simulink library "ASEToolBox2023a"  (R2023a)
settings: Solver=ode45  StartTime=0.0  StopTime=10.0  RelTol=1e-3  EnableMultiTasking=on
values from neighbouring files (symbols this model uses):
  dt = get_param(gcbh, 'g_output_datatype')    [maskSysComCallbacks_Receive.m]    (also in maskSysComCallbacks_Send.m = get_param(gcbh, 'g_input_datatype'))
undefined symbols (not defined in the file or in its folder): dCx, dCy, dCz, DiscIntNeverNeededParam, Discrete, dmassX, dmassY, dmassZ, dMx, dMy, dMz, dp, dp0, dp1, dp2, dp3, lmd_high, lmd_low, magnitude, Newton, p0, p1, p2, p3, p4, phi0, phi000, phi1, phi2, phi3, phi4, r1, r2, r3, r4, Raphson, theta0, theta1, theta2, theta3, theta4, Time, u0, u1, u2, u3, v0, v0_max, v0_min, v1, v111, v2, v222, v3, v333, v4, W1, w1, w2, W2 ... (+2)
libraries: simulink x38, etargetslib x28, simulink_extras x5, slpidlib x2, ctrlSharedLib x2, aerolibatmos2 x1, aerolibconvert2 x1, aerolibtransform2 x1, sharedtransform x1, dspstat3 x1, dspsolvers x1
(part 1 of 6)
settings Model: Creator=sunzx.fnst  LastModifiedBy=zqhkd
settings SolverCC: AlgebraicLoopSolver=TrustRegion
settings DataIOCC: LimitDataPoints=on  SaveFormat=Array  ReturnWorkspaceOutputs=off
settings OptimizationCC: LifeSpan=inf
settings DebuggingCC: UnderspecifiedInitializationDetection=Classic  MergeDetectMultiDrivingBlocksExec=none  SolverPrmCheckMsg=warning  UnconnectedInputMsg=warning  UnconnectedOutputMsg=warning  UnconnectedLineMsg=warning  SFUnexpectedBacktrackingDiag=warning  SFNoUnconditionalDefaultTransitionDiag=warning  SFExecutionAtInitializationDiag=none  ArithmeticOperatorsInVariantConditions=warning
settings HardwareCC: ProdBitPerPointer=32  ProdBitPerSizeT=32  ProdBitPerPtrDiffT=32  ProdLargestAtomicFloat=None  ProdIntDivRoundTo=Undefined  ProdEndianess=Unspecified  ProdWordSize=32  ProdHWDeviceType=32-bit Generic
settings ModelReferenceCC: PropagateSignalLabelsOutOfModel=off
settings SFSimCC: SimUseLocalCustomCode=off  CustomCodeUndefinedFunction=UseInterfaceOnly
settings RTWCC: RTWUseLocalCustomCode=off
settings CodeAppCC: StateflowObjectComments=on
settings GRTTargetCC: TargetLangStandard=C89/C90 (ANSI)
settings ConfigComp: CovMetricSettings=dw  CovSaveCumulativeToWorkspaceVar=on  CovSaveSingleToWorkspaceVar=on  CovExternalEMLEnable=off  CovSFcnEnable=off  CovBoundaryAbsTol=1.0e-5

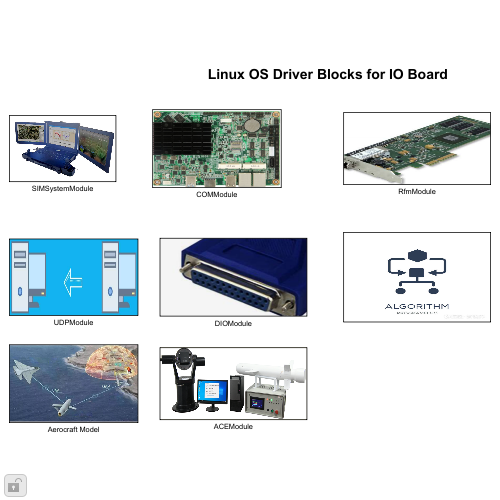
[thumbnail: Simulink's stored preview of the top-level diagram]
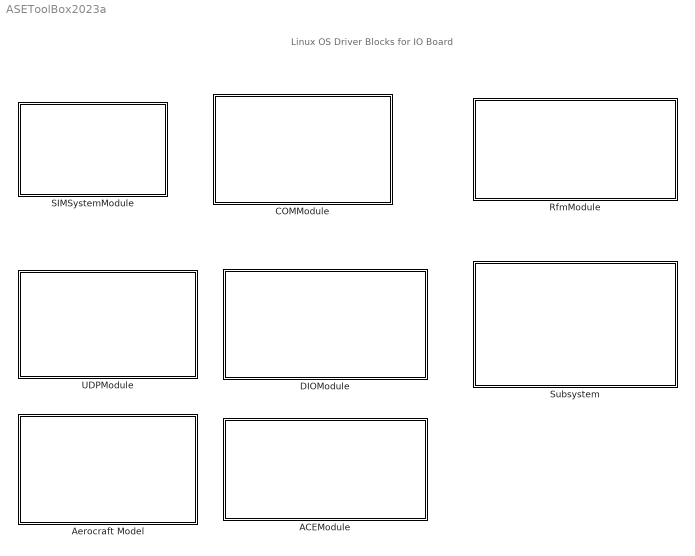
== system ASEToolBox2023a ==
  note: Linux OS Driver Blocks for IO Board
  ACEModule : Subsystem
      mask Display: image('ACEModule.png');
  Aerocraft Model : Subsystem
      mask Display: image('ASEApp.png');
  COMModule : Subsystem
      mask Display: image('MainBoardCom.png'); % 使用工具条上的 "编辑图像" 进行更改。
  DIOModule : Subsystem
      mask Display: image('parport.png'); % 使用工具条上的 "编辑图像" 进行更改。
  RfmModule : Subsystem
      mask Display: image('GE5565.png'); % 使用工具条上的 "编辑图像" 进行更改。
  SIMSystemModule : Subsystem
      mask Display: image('ASESystem.jpg'); % 使用工具条上的 "编辑图像" 进行更改。
  Subsystem : Subsystem
      mask Display: image('Algorithm.jpg'); % 使用工具条上的 "编辑图像" 进行更改。
  UDPModule : Subsystem
      mask Display: image('UDP.png'); % 使用工具条上的 "编辑图像" 进行更改。

== system ASEToolBox2023a/ACEModule ==
  IMU : Subsystem
  ServoCardPack : Subsystem  mask{g_FrameType=80, g_SendId=0}
      mask prompts: g_FrameType "请输入帧类型码："; g_SendId "发送方ID:"
      mask DialogControl ParameterGroupVar Prompt: 参数
  ServoCardUnpack : Subsystem
  TurnTable : Subsystem

== system ASEToolBox2023a/Aerocraft Model ==
  ACE Aerodynamic for 3DOF : Subsystem  mask(ACE Aerodynamic for 3DOF){}
      mask help: There is ACE Aerodynamic for 3DOF Model, including the ACE aircraft's aerodynamic force efficient models, and it is employed to simulate the 3DOF motion.
      mask Display:
      | %image(imread('aeroaerodynamics.bmp','bmp'),'center')
      | port_label('input',1,'Mach(M)','texmode','on');
      | port_label('input',2,'abv(deg)','texmode','on');
      | port_label('output',1,'Cxyz','texmode','on');
  ACE Aerodynamic for 6DOF : Subsystem  mask(ACE Aerodynamic for 6DOF){}
      mask help: There is ACE Aerodynamic for 6DOF Model, including the ACE aircraft's aerodynamic force efficient models and aerodynamic moment efficient models, and it is employed to simulate the 6DOF motion.
      mask Display:
      | %image(imread('aeroaerodynamics.bmp','bmp'),'center')
      | port_label('input',1,'Mach(M)','texmode','on');
      | port_label('input',2,'abv(deg)','texmode','on');
      | port_label('input',3,'WXYZ','texmode','on');
      | port_label('input',4,'Deltaxyz(deg)','texmode','on');
      | port_label('output',1,'Cxyz','texmode','on');
      | port_label('output',2,'mxyz','texmode','on');
  ACE Equation of 6DOF's Motion : Subsystem  mask(Equation of 6DOF's  Motion){}
      mask help: There is Equation of 6DOF Motion Model.
  ACE Guidance and Control Algorithm : Subsystem
  ACE Mass : Subsystem  mask(ACE Mass Properties){}
      mask help: There is ACE Mass Properties Model.
      mask Display:
      | %image(imread('aeromassprop.bmp','bmp'),'center');
      | port_label('input',1,'Time(s)','texmode','on');
      | port_label('output',1,'Mass(kg)','texmode','on');
  ACE Propulsion : Subsystem  mask(ACE Propulsion){}
      mask help: There is ACE Propulsion Model.
      mask Display:
      | %image(imread('aeropropulsion.bmp','bmp'),'center')
      | port_label('input',1,'Time(s)','texmode','on');
      | port_label('output',1,'P(N)','texmode','on');

== system ASEToolBox2023a/COMModule ==
  XComIn : S-Function  FunctionName=readXComAPI  Parameters=g_serial_select,g_baudrate, g_parity, g_databit, g_stopbit, g_data_size, g_sample_time  SFunctionDeploymentMode=off  EnableBusSupport=off  mask(CP-116E-A接收模块){g_serial_select=ttyMUE0, g_baudrate=460800, g_parity=None, g_databit=8, g_stopbit=1, g_data_size=1, g_sample_time=-1}
      mask prompts: g_serial_select "串口号："; g_baudrate "波特率："; g_parity "校验位："; g_databit "数据位："; g_stopbit "停止位："; g_data_size "帧长度："; g_sample_time "采样时间："
      mask help:
      | 多串口中选择串口号的数据接收模块。
      | 用户需要指定串口设备号、接收数据的数据类型和长度。
      | 串口接收模块有两个输出端口，第一个端口输出串口上发来被接收到的数据，并转换为用户设定的数据类型发出；
      | 第二个端口Len表示每个步长下所接收到的数据长度，用于帮助用户分析和对数据进行后处理。
      mask Help: https://moxa.com.cn/products/industrial-edge-connectivity/multiport-serial-boards/pcie-upci-pci-serial-cards/cp-116e-a
      mask TypeOptions g_serial_select: ttyS0 | ttyS1 | ttyS2 | ttyS3 | ttyS4 | ttyS5 | ttyS6 | ttyMUE0 | ttyMUE1 | ttyMUE2 | ttyMUE3 | ttyMUE4 | ttyMUE5 | ttyMUE6 | ttyMUE7 | ttyMUE8 | ttyMUE9 | ttyMUE10 | ttyMUE11 | ttyMUE12 | ttyMUE13 | ttyMUE14 | ttyMUE15 | ttyUSB0 | ttyUSB1 | ttyUSB2 | ttyUSB3 | Custom
      mask TypeOptions g_baudrate: 921600 | 576000 | 500000 | 460800 | 230400 | 115200 | 57600 | 38400 | 19200 | 9600 | Custom
      mask TypeOptions g_parity: None | Odd | Even | Mark | Space
      mask DialogControl ParameterGroupVar Prompt: ASE仿真系统串口接收模块
      mask Display:
      | color('blue');
      | serialDevice = get_param(gcbh, 'g_serial_select');
      | port_label('output', 1, serialDevice);
      | image('MainBoardCom.png', [0 0 0.33 0.48]);
  XComOut : S-Function  FunctionName=writeXComAPI  Parameters=g_serial_select,g_baudrate, g_parity, g_databit, g_stopbit,g_sample_time  SFunctionDeploymentMode=off  EnableBusSupport=off  mask(CP-116E-A发送模块){g_serial_select=ttyMUE0, g_baudrate=460800, g_parity=None, g_databit=8, g_stopbit=1, g_sample_time=-1}
      mask prompts: g_serial_select "串口号："; g_baudrate "波特率："; g_parity "校验位："; g_databit "数据位："; g_stopbit "停止位："; g_sample_time "采样时间："
      mask help: 根据用户设置的串口号，指定的数据类型，将数据对外部进行发送的模块。
      mask Help: https://moxa.com.cn/products/industrial-edge-connectivity/multiport-serial-boards/pcie-upci-pci-serial-cards/cp-116e-a
      mask TypeOptions g_serial_select: ttyS0 | ttyS1 | ttyS2 | ttyS3 | ttyS4 | ttyS5 | ttyS6 | ttyMUE0 | ttyMUE1 | ttyMUE2 | ttyMUE3 | ttyMUE4 | ttyMUE5 | ttyMUE6 | ttyMUE7 | ttyMUE8 | ttyMUE9 | ttyMUE10 | ttyMUE11 | ttyMUE12 | ttyMUE13 | ttyMUE14 | ttyMUE15 | ttyUSB0 | ttyUSB1 | ttyUSB2 | ttyUSB3 | Custom
      mask TypeOptions g_baudrate: 921600 | 576000 | 500000 | 460800 | 230400 | 115200 | 57600 | 38400 | 19200 | 9600 bps
      mask TypeOptions g_parity: None | Odd | Even | Mark | Space
      mask DialogControl ParameterGroupVar Prompt: ASE仿真串口发送模块
      mask Display:
      | color('blue');
      | serialDevice = get_param(gcbh, 'g_serial_select');
      | port_label('input', 1, serialDevice);
      | image('MainBoardCom.png', [0.67 0 1.0 0.48]);

== system ASEToolBox2023a/DIOModule ==
  ParPortRead : S-Function  FunctionName=ParPortDataRead  Parameters=g_par_select, g_ext_trigger, g_pin  SFunctionDeploymentMode=off  EnableBusSupport=off  mask(Linux工控机主板并口设备){g_par_select=/dev/parport0, g_ext_trigger=on, g_pin=PIN15 (S3)}
      mask prompts: g_par_select "并口设备号:"; g_ext_trigger "外部时钟源触发:"; g_pin "时钟源PIN:"
      mask help: 此模块将输出Linux IPC并口设备的数据寄存器的值。数据寄存器包括D7|D6|D5|D4|D3|D2|D1|D0总共8个数据位，合并位uint8类型输出。
      mask TypeOptions g_par_select: /dev/parport0
      mask TypeOptions g_pin: PIN15 (S3) | PIN13 (S4) | PIN12 (S5) | PIN10 (S6) | PIN11 (S7)
      mask DialogControl ParameterGroupVar Prompt: 工控机主板板载并口管理
      mask DialogControl Control1 Prompt: 此模块将输出工控机主板并口设备DB25输入引脚高低电平状态。各引脚和输入寄存器位之间关系如下：
      mask DialogControl Control3 Prompt: P15--Di3, P13--Di4, P12--Di5, P10--Di6, P11--Di7
      mask DialogControl g_pin Tooltip: 并口DB25引脚定义
      mask Display:
      | warning off;
      | image('parport.png');
      | ext_trigger = get_param(gcbh, 'g_ext_trigger');
      | pin = get_param(gcbh, 'g_pin');
      | if strcmp(ext_trigger, 'off')
      |     color('cyan');
      |     port_label('output', 1, 'data');
      | else
      |     color('cyan');
      |     disp(['外部时钟源:' pin]);
      | end
  ParPortWrite : S-Function  FunctionName=ParPortDataWrite  Parameters=g_par_select  SFunctionDeploymentMode=off  EnableBusSupport=off  mask(Linux工控机主板并口设备){g_par_select=/dev/parport0}
      mask prompts: g_par_select "并口号:"
      mask help: 此模块将模型输入值写入到Linux IPC并口设备的数据寄存器。数据寄存器包括D7|D6|D5|D4|D3|D2|D1|D0总共8个数据位，模型中将8个bit合并为uint8类型输入。
      mask TypeOptions g_par_select: /dev/parport0
      mask DialogControl ParameterGroupVar Prompt: 工控机并口管理模块
      mask DialogControl Control1 Prompt: 此模块将从工控机主板并口设备DB25对应引脚上输出信号的高低电平值。各引脚和输出寄存器位之间关系如下：
      mask DialogControl Control2 Prompt: P2 -Do0, P3--Do1, P4--Do2, P5--Do3, P6--Do4,P7--Do5,P8--Do6,P9--Do7
      mask Display:
      | image('parport.png');
      | %color('blue');
      | %dio = get_param(gcbh, 'g_par_select');
      | %disp(dio);
      | color('cyan');
      | port_label('input', 1, 'data');

== system ASEToolBox2023a/RfmModule ==
  RFM2gInit : S-Function  FunctionName=RFM2gInit_sfcn  SFunctionDeploymentMode=off  EnableBusSupport=off  mask(GE5565反射内存卡初始化模块){}
      mask help:
      | 软件启动时，初始化中使用RFM2gOpen()启动反射内存设备；
      | 软件终止时，终止回调中使用RFM2gClose()关闭反射内存设备。
      mask DialogControl ParameterGroupVar Prompt: 参数
      mask Display:
      | color('blue');
      | disp('Devce: /dev/rfm2g0');
      | image('GE5565.png',[0 0 0.3 0.4]); % 使用工具条上的 "编辑图像" 进行更改。
  RFM2gRead : S-Function  FunctionName=RFM2gRead_sfcn  Parameters=g_datatype, g_base_addr, g_offset, g_length, g_sample_time  SFunctionDeploymentMode=off  EnableBusSupport=off  mask(GE5565反射内存读模块){g_datatype=double, g_base_addr=0x00000000, g_offset=0, g_length=1, g_sample_time=0.01}
      mask prompts: g_datatype "数据类型:"; g_base_addr "基地址:"; g_offset "偏移量:"; g_length "读取长度:"; g_sample_time "采样时间:"
      mask help:
      | GE5565反射内存读模块，根据模型设置，针对偏移地址读取指定数据类型和指定长度的数据。
      | 总的偏移量为基地址+偏移量；
      | 读取长度至少是1，可以根据用户指定的数据类型自适应读取存储区域的大小范围。
      mask TypeOptions g_datatype: double | single | int8 | uint8 | int16 | uint16 | int32 | uint32 | boolean
      mask DialogControl ParameterGroupVar Prompt: 参数
      mask Display:
      | %port_label('output', 1, 'data');
      | color('blue');
      | datatype = get_param(gcbh, 'g_datatype');
      | offset = get_param(gcbh, 'g_offset');
      | disp(['Datatype: ' datatype newline 'Offset: ' num2str(offset)]);
      | image('GE5565.png',[0 0 0.3 0.4]); % 使用工具条上的 "编辑图像" 进行更改。
  RFM2gWrite : S-Function  FunctionName=RFM2gWrite_sfcn  Parameters=g_datatype, g_base_addr, g_offset, g_sample_time  SFunctionDeploymentMode=off  EnableBusSupport=off  mask(GE_5565反射内存写入模块){g_datatype=double, g_base_addr=0x00000000, g_offset=0, g_sample_time=0.001}
      mask prompts: g_datatype "数据类型:"; g_base_addr "基地址:"; g_offset "偏移量:"; g_sample_time "采样时间:"
      mask help: GE_5565反射内存写入模块，针对输入信号的数据类型进行配置，并根据用户协议设置基地址和偏移量Offset后使用。
      mask Help: https://blog.csdn.net/trueleven/article/details/7729039
      mask TypeOptions g_datatype: double | single | int8 | uint8 | int16 | uint16 | int32 | uint32 | boolean
      mask Display:
      | %port_label('input', 1, 'data');
      | color('blue');
      | datatype = get_param(gcbh, 'g_datatype');
      | offset = get_param(gcbh, 'g_offset');
      | disp(['Datatype: ' datatype newline 'Offset: ' num2str(offset)]);
      | image('GE5565.png',[0 0 0.3 0.4]); % 使用工具条上的 "编辑图像" 进行更改。

== system ASEToolBox2023a/SIMSystemModule ==
  ASEMonitorIn : Subsystem  mask{g_iVarNum=1, g_iFrameType=10, g_ip="192.168.0.3", g_sample_time=0.01, g_buffersize=16}
      mask prompts: g_iVarNum "请输入监测数据维度："; g_iFrameType "请输入帧类型码："; g_ip "请输入上位机IP地址："; g_sample_time "请输入采样时间："; g_buffersize "缓冲区大小计算值（字节)："
      mask DialogControl ParameterGroupVar Prompt: ASE监控台注入管理窗口
      mask DialogControl g_iVarNum Tooltip: 注意每个信号对应一个4字节的single类型单精度浮点数
      mask DialogControl g_buffersize Tooltip: UDP传输时缓冲区长度为varNum*4 + 12字节
      mask DialogControl Control1 Prompt: 请进行信号名称校验
      mask Display:
      | ip = get_param(gcb, 'g_ip');
      | color('blue');
      | disp(['MonitorIP' newline ip]);
  ASEMonitorOut : Subsystem  Tag=ASEMonitorOutTag  mask{g_iVarNum=1, g_iFrameType=10, g_hostIP="192.168.0.3", g_buffersize=16}
      mask prompts: g_iVarNum "请输入监测信号维度："; g_iFrameType "请输入帧类型码："; g_hostIP "请输入上位机IP地址："; g_buffersize "缓冲区大小计算值（字节)："
      mask DialogControl ParameterGroupVar Prompt: 监测信号参数管理窗口
      mask DialogControl g_iVarNum Tooltip: 注意每个信号对应一个4字节的single类型单精度浮点数
      mask DialogControl g_buffersize Tooltip: UDP传输时缓冲区长度为varNum*4 + 12字节
      mask DialogControl Control1 Prompt: 校验监测信号名称
      mask Display:
      | ip = get_param(gcb, 'g_hostIP');
      | color('blue');
      | disp(['MonitorIP' newline ip]);
  ASETimer : S-Function  Priority=0  FunctionName=aseSimTimer  Parameters=g_sampleTime  SFunctionDeploymentMode=off  EnableBusSupport=off  mask{g_sampleTime=0.002}
      mask prompts: g_sampleTime "请输入采样时间："
      mask DialogControl DescGroupVar Prompt: ASETarget仿真机时钟获取模块
      mask DialogControl Control2 Prompt: 本模块能够直接访问ASE仿真系统运行时间，起始点为仿真开始时间，单位为秒。
      mask Display: color('gray');port_label('output',1,'Tim /s');

== system ASEToolBox2023a/Subsystem ==
  Formation-Control : Subsystem  mask{theta0=theta0, phi0=phi0, v0=v0, p0=p0, theta1=theta1, phi1=phi1, v1=v1, p1=p1, r1=r1, theta2=theta2, phi2=phi2, v2=v2, p2=p2, r2=r2, theta3=theta3, phi3=phi3, v3=v3, p3=p3, r3=r3, theta4=theta4, phi4=phi4, v4=v4, p4=p4, r4=r4, dp0=dp0, dp1=dp1, dp2=dp2, dp3=dp3}
      mask prompts: theta0 "Leader-Initial theta"; phi0 "Leader-Initial phi"; v0 "Leader-Initial v"; p0 "Leader-Initial p"; theta1 "Follower1-Initial theta"; phi1 "Follower1-Initial phi"; v1 "Follower1-Initial v"; p1 "Follower1-Initial p"; r1 "Follower1-Initial r"; theta2 "Follower2-Initial theta"; phi2 "Follower2-Initial phi"; v2 "Follower2-Initial v"; p2 "Follower2-Initial p"; r2 "Follower2-Initial r"; theta3 "Follower3-Initial theta"; phi3 "Follower3-Initial phi"; v3 "Follower3-Initial v"; p3 "Follower3-Initial p"; r3 "Follower3-Initial r"; theta4 "Follower4-Initial theta"; phi4 "Follower4-Initial phi"; v4 "Follower4-Initial v"; p4 "Follower4-Initial p"; r4 "Follower4-Initial r"; dp0 "Follower1"; dp1 "Follower2"; dp2 "Follower3"; dp3 "Follower4"
      mask DialogControl DescGroupVar Prompt: Leader初始参数
      mask DialogControl ParameterGroupVar Prompt: Follower初始参数
      mask DialogControl Container4 Prompt: Follower1
      mask DialogControl ParameterGroupVar_copy_copy_copy Prompt: Follower2
      mask DialogControl ParameterGroupVar_copy_copy_copy_copy Prompt: Follower3
      mask DialogControl ParameterGroupVar_copy_copy_copy_copy_copy Prompt: Follower4
      mask DialogControl Container7 Prompt: 相对Leader几何关系
  GNC_EKF : Subsystem  mask{dt=0.002}
      mask prompts: dt "步长"
      mask DialogControl ParameterGroupVar Prompt: 参数

== system ASEToolBox2023a/UDPModule ==
  UDP_Receive : S-Function  Priority=6  FunctionName=UDPRecv_sfcn  Parameters=g_localip, g_localport, g_ip, g_port, g_buffersize, g_datatype, g_sample_time,g_reusePort  SFunctionDeploymentMode=off  EnableBusSupport=off  mask(UDP Receive){g_localip="192.168.0.7", g_localport=8080, g_ip="192.168.0.3", g_port=9090, g_buffersize=8, g_datatype=double, g_sample_time=0.01, g_reusePort=0}
      mask prompts: g_localip "本机IP地址:"; g_localport "端口号:"; g_ip "远程IP地址:"; g_port "远程端口号:"; g_buffersize "接收缓存大小:"; g_datatype "数据类型:"; g_sample_time "采样时间:"; g_reusePort "收发是否都用同一个端口:"
      mask help:
      | Receive UDP packets on the host computer at the specified local port.
      |
      | The block outputs the received UDP data as a one-dimensional array of the specified data type.
      |
      | Set the Local IP port parameter to the desired port where the sender sends the UDP data. Set the Data type parameter to match the data type of the incoming UDP data. Set the Blocking time parameter to specify the duration to wait for a UDP packet before continuing.
      |
      | 注意：IP请使用双引号括起来，如"192.168.0.7"。
      mask TypeOptions g_datatype: double | single | int8 | uint8 | int16 | uint16 | int32 | uint32 | boolean
      mask DialogControl ParameterGroupVar Prompt: 参数
      mask Display:
      | port_label('output', 1, 'Data');
      | port_label('output', 2, 'Len');
      | ip = get_param(gcb, 'g_ip');
      | port = get_param(gcb, 'g_port');
      | color('blue');
      | disp(['UDP Receive' newline 'IP:' ip newline 'Port:' port]);
  UDP_Send : S-Function  Priority=0  FunctionName=UDPSend_sfcn  Parameters=g_localIP, g_localPort, g_ip, g_port, g_buffersize  SFunctionDeploymentMode=off  EnableBusSupport=off  mask(UDP Send){g_localIP="192.168.0.7", g_localPort=8080, g_ip="192.168.0.3", g_port=9090, g_buffersize=8}
      mask prompts: g_localIP "本机IP地址:"; g_localPort "本机端口:"; g_ip "远程机IP地址:"; g_port "远程机端口号:"; g_buffersize "发送缓存大小:"
      mask help: Send a UDP packet to a network address identified by the remote IP address and remote IP port parameters.
      mask DialogControl ParameterGroupVar Prompt: 参数
      mask Display:
      | port_label('input', 1, 'Data');
      | ip = get_param(gcb, 'g_ip');
      | port = get_param(gcb, 'g_port');
      | color('blue');
      | disp(['UDP Send' newline 'IP:' ip newline 'Port:' port]);

== system ASEToolBox2023a/ACEModule/IMU ==
  AFCCom : Inport
  Demux : Demux  Outputs=[3,3]
  FrameCheck3 : Subsystem
  Subsystem5 : Subsystem
  Terminator : Terminator
  Terminator1 : Terminator
  Terminator2 : Terminator
  Wxyz : Outport
  Axyz : Outport  Port=2
  wires:
  Subsystem5/2(SourceID) -> Terminator1/1
  FrameCheck3/1(Out1) -> Subsystem5/Enable
  AFCCom/1 -> FrameCheck3/1(In1), Subsystem5/1(In1)
  Subsystem5/1(Counter) -> Terminator/1  "AFC_ACK_COUNTER"
  Subsystem5/3(FrameType) -> Terminator2/1
  Subsystem5/4(Para) -> Demux/1
  Demux/1 -> Wxyz/1
  Demux/2 -> Axyz/1

== system ASEToolBox2023a/ACEModule/ServoCardPack ==
  Parms : Inport
  BitChk : Subsystem
  Byte Pack10 : etargetslib/Byte Pack  datatypes={'uint16'}  byteAlign=1
  Byte Pack3 : etargetslib/Byte Pack  datatypes={'uint16'}  byteAlign=1
  Byte Pack6 : etargetslib/Byte Pack  datatypes={'uint32'}  byteAlign=1
  Byte Pack7 : etargetslib/Byte Pack  datatypes={'uint16'}  byteAlign=1
  Byte Pack8 : etargetslib/Byte Pack  datatypes={'single'}  byteAlign=1
  Constant3 : Constant  Value=0xDAA5
  Data Type Conversion4 : DataTypeConversion  OutDataTypeStr=uint16  SaturateOnIntegerOverflow=off  RndMeth=Floor
  Data Type Conversion5 : DataTypeConversion  OutDataTypeStr=uint16  SaturateOnIntegerOverflow=off  RndMeth=Floor
  Data Type Conversion6 : DataTypeConversion  OutDataTypeStr=uint32  SaturateOnIntegerOverflow=off  RndMeth=Floor
  Data Type Conversion7 : DataTypeConversion  OutDataTypeStr=uint8  SaturateOnIntegerOverflow=off  RndMeth=Floor
  Data Type Conversion8 : DataTypeConversion  OutDataTypeStr=single  SaturateOnIntegerOverflow=off  RndMeth=Floor
  Data Type Conversion9 : DataTypeConversion  OutDataTypeStr=uint16  SaturateOnIntegerOverflow=off  RndMeth=Floor
  FrameTimeTick : simulink/Sources/Counter Free-Running  NumBits=32  tsamp=-1
  FrameTypeCode : Constant  Value=g_FrameType
  ID : Constant  Value=g_SendId
  Mux2 : Mux  Inputs=6
  Mux3 : Mux  Inputs=2
  Signal Copy2 : SignalConversion  OverrideOpt=on
  Width2 : Width  DataType=single
  SrvoCard : Outport
  wires:
  Data Type Conversion5/1 -> Byte Pack3/1
  Constant3/1 -> Data Type Conversion9/1
  ID/1 -> Data Type Conversion4/1
  Width2/1 -> Data Type Conversion5/1
  Mux2/1 -> BitChk/1(In1), Mux3/1
  Data Type Conversion7/1 -> Mux2/5
  Data Type Conversion4/1 -> Byte Pack7/1
  Byte Pack3/1 -> Mux2/2
  Byte Pack8/1 -> Mux2/6
  Byte Pack6/1 -> Mux2/3
  FrameTimeTick/1 -> Data Type Conversion6/1  "AseCounter"
  Data Type Conversion6/1 -> Byte Pack6/1
  Data Type Conversion8/1 -> Byte Pack8/1
  Data Type Conversion9/1 -> Byte Pack10/1
  Mux3/1 -> Width2/1, Signal Copy2/1
  Byte Pack7/1 -> Mux2/4
  FrameTypeCode/1 -> Data Type Conversion7/1
  BitChk/1(Out1) -> Mux3/2
  Byte Pack10/1 -> Mux2/1
  Parms/1 -> Data Type Conversion8/1
  Signal Copy2/1 -> SrvoCard/1

== system ASEToolBox2023a/ACEModule/ServoCardUnpack ==
  SrvoCard : Inport
  FrameCheck1 : Subsystem
  Subsystem6 : Subsystem
  Terminator1 : Terminator
  Terminator2 : Terminator
  Parms : Outport
  FrameTick : Outport  Port=2
  wires:
  Subsystem6/2(ACKSourceID) -> Terminator1/1
  Subsystem6/1(ACKFrameCounter) -> FrameTick/1  "AFC_ACK_COUNTER"
  FrameCheck1/1(Out1) -> Subsystem6/Enable
  Subsystem6/4(ACKFramePara) -> Parms/1
  SrvoCard/1 -> FrameCheck1/1(In1), Subsystem6/1(In1)
  Subsystem6/3(ACKFrameType) -> Terminator2/1

== system ASEToolBox2023a/ACEModule/TurnTable ==
  X : Inport
  Y : Inport  Port=2
  Z : Inport  Port=3
  8BitCheckSum1 : Subsystem
  Byte Pack1 : etargetslib/Byte Pack  datatypes={'int32'}  byteAlign=1
  Byte Pack12 : etargetslib/Byte Pack  datatypes={'uint8'}  byteAlign=1
  Byte Pack13 : etargetslib/Byte Pack  datatypes={'uint8'}  byteAlign=1
  Byte Pack14 : etargetslib/Byte Pack  datatypes={'uint8'}  byteAlign=1
  Byte Pack2 : etargetslib/Byte Pack  datatypes={'int32'}  byteAlign=1
  Byte Pack4 : etargetslib/Byte Pack  datatypes={'uint16'}  byteAlign=1
  Byte Pack5 : etargetslib/Byte Pack  datatypes={'int32'}  byteAlign=1
  Constant : Constant  Value=32
  Constant4 : Constant  Value=0xDAA5
  CounterFreeRunning1 : simulink/Sources/Counter Free-Running  NumBits=8  tsamp=-1
  Data Type Conversion1 : DataTypeConversion  OutDataTypeStr=int32  SaturateOnIntegerOverflow=off  RndMeth=Floor
  Data Type Conversion{10..12,14,18} (5 alike) : DataTypeConversion  OutDataTypeStr=uint8  SaturateOnIntegerOverflow=off  RndMeth=Floor
  Data Type Conversion17 : DataTypeConversion  OutDataTypeStr=uint16  SaturateOnIntegerOverflow=off  RndMeth=Floor
  Data Type Conversion2 : DataTypeConversion  OutDataTypeStr=int32  SaturateOnIntegerOverflow=off  RndMeth=Floor
  Data Type Conversion3 : DataTypeConversion  OutDataTypeStr=int32  SaturateOnIntegerOverflow=off  RndMeth=Floor
  Gain : Gain  Gain=5000
  Gain1 : Gain  Gain=5000
  Gain2 : Gain  Gain=5000
  Mux : Mux  Inputs=9
  Mux4 : Mux  Inputs=2
  Saturation : Saturate  UpperLimit=3600  LowerLimit=-3600
  Saturation1 : Saturate  UpperLimit=3600  LowerLimit=-3600
  Saturation2 : Saturate  UpperLimit=3600  LowerLimit=-3600
  Signal Copy1 : SignalConversion  OverrideOpt=on
  Width1 : Width  DataType=single
  Frame : Outport
  wires:
  Mux4/1 -> Width1/1, Signal Copy1/1
  Byte Pack1/1 -> Mux/8
  Data Type Conversion2/1 -> Byte Pack1/1
  Saturation1/1 -> Gain1/1
  Data Type Conversion17/1 -> Byte Pack4/1
  8BitCheckSum1/1(Out1) -> Mux4/2
  X/1 -> Saturation/1  "XPosVell_Com"
  Byte Pack5/1 -> Mux/7
  Z/1 -> Saturation2/1  "ZPosVell_Com"
  Data Type Conversion10/1 -> Mux/2
  Constant/1 -> Data Type Conversion14/1, Data Type Conversion12/1, Data Type Conversion18/1  "Zmode"
  Byte Pack13/1 -> Mux/6
  Data Type Conversion12/1 -> Byte Pack12/1
  Width1/1 -> Data Type Conversion10/1
  Mux/1 -> 8BitCheckSum1/1(In1), Mux4/1
  Byte Pack4/1 -> Mux/1
  Byte Pack14/1 -> Mux/4
  Data Type Conversion11/1 -> Mux/3
  Byte Pack2/1 -> Mux/9
  Saturation2/1 -> Gain2/1
  Data Type Conversion1/1 -> Byte Pack5/1
  Data Type Conversion3/1 -> Byte Pack2/1
  Saturation/1 -> Gain/1
  Constant4/1 -> Data Type Conversion17/1
  Data Type Conversion18/1 -> Byte Pack14/1
  Data Type Conversion14/1 -> Byte Pack13/1
  Gain1/1 -> Data Type Conversion2/1
  Y/1 -> Saturation1/1  "YPosVell_Com"
  Byte Pack12/1 -> Mux/5
  Gain/1 -> Data Type Conversion1/1
  Gain2/1 -> Data Type Conversion3/1
  CounterFreeRunning1/1 -> Data Type Conversion11/1  "AseCounter"
  Signal Copy1/1 -> Frame/1

== system ASEToolBox2023a/Aerocraft Model/ACE Aerodynamic for 3DOF ==
  Ma : Inport
  abv : Inport  Port=2
  CD : Lookup2D  RowIndex=[-2 -1 0.5 1 2 3 4 5 6 7 8 9 10]  ColumnIndex=[0.3 0.4 0.5 0.6 0.7 0.8]  Table=|  SaturateOnIntegerOverflow=off  InputSameDT=off
      | [0.184400000000000	0.176300000000000	0.168500000000000	0.162600000000000	0.158700000000000	0.154800000000000
      | 0.194000000000000	0.185600000000000	0.177400000000000	0.171100000000000	0.166800000000000	0.162200000000000
      | 0.196300000000000	0.187800000000000	0.179600000000000	0.173200000000000	0.168700000000000	0.164000000000000
      | 0.194000000000000	0.185600000000000	0.177400000000000	0.171100000000000	0.166800000000000	0.162200000000000
      | 0.184400000000000	0.176300000000000	0.168500000000000	0.162600000000000	0.158700000000000	0.154800000000000
      | 0.168000000000000	0.160300000000000	0.153000000000000	0.147900000000000	0.144800000000000	0.141900000000000
      | 0.144500000000000	0.137300000000000	0.130800000000000	0.126700000000000	0.124700000000000	0.123200000000000
      | 0.113500000000000	0.107100000000000	0.101600000000000	0.0987000000000000	0.0982000000000000	0.0985000000000000
      | 0.0748000000000000	0.0694000000000000	0.0651000000000000	0.0637000000000000	0.0650000000000000	0.0674000000000000
      | 0.0284000000000000	0.0241000000000000	0.0212000000000000	0.0217000000000000	0.0250000000000000	0.0300000000000000
      | -0.0258000000000000	-0.0289000000000000	-0.0302000000000000	-0.0276000000000000	-0.0220000000000000	-0.0140000000000000
      | -0.0878000000000000	-0.0895000000000000	-0.0890000000000000	-0.0841000000000000	-0.0758000000000000	-0.0646000000000000
      | -0.157700000000000	-0.157800000000000	-0.155300000000000	-0.147900000000000	-0.136600000000000	-0.121800000000000
      | ]
  CL : Subsystem
  DeltZ_pp : Lookup2D  RowIndex=|  ColumnIndex=|  Table=|  SaturateOnIntegerOverflow=off  InputSameDT=off
      RowIndex=|
      | [-2
      | -1
      | 0.5
      | 1
      | 2
      | 3
      | 4
      | 5
      | 6
      | 7
      | 8
      | 9
      | 10
      | ]
      Table=|
      | [-3.41201716738197	-3.29113924050633	-3.14937759336100	-2.95934959349594	-2.79268292682927	-2.53658536585366
      | -1.70386266094421	-1.64556962025316	-1.56611570247934	-1.47967479674797	-1.39430894308943	-1.26829268292683
      | 0.854077253218884	0.822784810126582	0.780991735537190	0.739837398373984	0.699186991869919	0.634146341463415
      | 1.70386266094421	1.64556962025316	1.56611570247934	1.47967479674797	1.39430894308943	1.26829268292683
      | 3.41201716738197	3.29113924050633	3.14937759336100	2.95934959349594	2.79268292682927	2.53658536585366
      | 5.14224137931035	4.93670886075949	4.72199170124481	4.45714285714286	4.20816326530612	3.82448979591837
      | 6.84913793103448	6.60169491525424	6.31666666666667	5.93877551020408	5.60816326530612	5.09795918367347
      | 8.58441558441558	8.27659574468085	7.88333333333333	7.44262295081967	7.03278688524590	6.38934426229508
      | 10.3260869565217	9.95299145299145	9.48117154811716	8.95061728395062	8.46090534979424	7.69135802469136
      | 12.0655021834061	11.6309012875536	11.0798319327731	10.4586776859504	9.88842975206612	8.99173553719008
      | 13.7982456140351	13.3017241379310	12.7245762711864	11.9626556016598	11.3112033195021	10.2904564315353
      | 15.5198237885463	14.9610389610390	14.3148936170213	13.5146443514644	12.7824267782427	11.6317991631799
      | 17.3066666666667	16.6812227074236	15.9570815450644	15.0084033613445	14.1932773109244	12.9243697478992
      | ]
      ColumnIndex=|
      | [0.3	0.4	0.5	0.6	0.7	0.8
      | ]
  Mux : Mux  Inputs=3
  Selector : Selector  InputPortWidth=3  IndexOptions=Index vector (dialog)  Indices=[1]  OutputSizes=1
  Selector1 : Selector  InputPortWidth=3  IndexOptions=Index vector (dialog)  Indices=[2]  OutputSizes=1
  Subsystem1 : Subsystem
  Cxyz : Outport
  wires:
  Subsystem1/1(CZ) -> Mux/3
  CL/1(CL) -> Mux/2
  CD/1 -> Mux/1
  Mux/1 -> Cxyz/1
  Selector1/1 -> Subsystem1/1(beta)  "beta"
  Selector/1 -> CD/1, CL/1(alpha), DeltZ_pp/1, Subsystem1/2(alpha)  "alpha"
  abv/1 -> Selector1/1, Selector/1
  Ma/1 -> CD/2, CL/2(Ma), DeltZ_pp/2, Subsystem1/3(Ma)  "Ma"
  DeltZ_pp/1 -> CL/3(deltz_pp)

== system ASEToolBox2023a/Aerocraft Model/ACE Aerodynamic for 6DOF ==
  Ma : Inport
  abv : Inport  Port=2
  WXYZ : Inport  Port=3
  DeltXYZ : Inport  Port=4
  CD : Lookup2D  RowIndex=[-2 -1 0.5 1 2 3 4 5 6 7 8 9 10]  ColumnIndex=[0.3 0.4 0.5 0.6 0.7 0.8]  Table=|  SaturateOnIntegerOverflow=off  InputSameDT=off
      | [0.184400000000000	0.176300000000000	0.168500000000000	0.162600000000000	0.158700000000000	0.154800000000000
      | 0.194000000000000	0.185600000000000	0.177400000000000	0.171100000000000	0.166800000000000	0.162200000000000
      | 0.196300000000000	0.187800000000000	0.179600000000000	0.173200000000000	0.168700000000000	0.164000000000000
      | 0.194000000000000	0.185600000000000	0.177400000000000	0.171100000000000	0.166800000000000	0.162200000000000
      | 0.184400000000000	0.176300000000000	0.168500000000000	0.162600000000000	0.158700000000000	0.154800000000000
      | 0.168000000000000	0.160300000000000	0.153000000000000	0.147900000000000	0.144800000000000	0.141900000000000
      | 0.144500000000000	0.137300000000000	0.130800000000000	0.126700000000000	0.124700000000000	0.123200000000000
      | 0.113500000000000	0.107100000000000	0.101600000000000	0.0987000000000000	0.0982000000000000	0.0985000000000000
      | 0.0748000000000000	0.0694000000000000	0.0651000000000000	0.0637000000000000	0.0650000000000000	0.0674000000000000
      | 0.0284000000000000	0.0241000000000000	0.0212000000000000	0.0217000000000000	0.0250000000000000	0.0300000000000000
      | -0.0258000000000000	-0.0289000000000000	-0.0302000000000000	-0.0276000000000000	-0.0220000000000000	-0.0140000000000000
      | -0.0878000000000000	-0.0895000000000000	-0.0890000000000000	-0.0841000000000000	-0.0758000000000000	-0.0646000000000000
      | -0.157700000000000	-0.157800000000000	-0.155300000000000	-0.147900000000000	-0.136600000000000	-0.121800000000000
      | ]
  CL Subsystem : Subsystem
  CZ Subsystem : Subsystem
  Mux : Mux  Inputs=3
  Mux1 : Mux  Inputs=3
  Mx Subsystem : Subsystem
  My Subsystem : Subsystem
  Mz Subsystem : Subsystem
  Selector : Selector  InputPortWidth=3  IndexOptions=Index vector (dialog)  Indices=[1]  OutputSizes=1
  Selector1 : Selector  InputPortWidth=3  IndexOptions=Index vector (dialog)  Indices=[2]  OutputSizes=1
  Selector2 : Selector  InputPortWidth=3  IndexOptions=Index vector (dialog)  Indices=[1]  OutputSizes=1
  Selector3 : Selector  InputPortWidth=3  IndexOptions=Index vector (dialog)  Indices=[1]  OutputSizes=1
  Selector4 : Selector  InputPortWidth=3  IndexOptions=Index vector (dialog)  Indices=[2]  OutputSizes=1
  Selector5 : Selector  InputPortWidth=3  IndexOptions=Index vector (dialog)  Indices=3  OutputSizes=1
  Selector6 : Selector  InputPortWidth=3  IndexOptions=Index vector (dialog)  Indices=3  OutputSizes=1
  Cxyz : Outport
  Mxyz : Outport  Port=2
  wires:
  Selector6/1 -> Mz Subsystem/3(DeltZ), CL Subsystem/3(DeltZ)  "DeltZ"
  Selector5/1 -> Mz Subsystem/4(WZ)  "WZ"
  Selector4/1 -> Mx Subsystem/6(WY), My Subsystem/3(WY)  "WY"
  Selector3/1 -> My Subsystem/2(WX), Mx Subsystem/5(WX)  "WX"
  Selector2/1 -> Mx Subsystem/4(DeltX)  "DeltX"
  WXYZ/1 -> Selector5/1, Selector4/1, Selector3/1
  DeltXYZ/1 -> Selector6/1, Selector2/1
  Mz Subsystem/1(Mz) -> Mux1/3
  Ma/1 -> Mz Subsystem/1(Ma), My Subsystem/4(Ma), Mx Subsystem/2(Ma), CZ Subsystem/3(Ma), CL Subsystem/2(Ma), CD/2  "Ma"
  abv/1 -> Selector/1, Selector1/1
  CD/1 -> Mux/1
  CL Subsystem/1(CL) -> Mux/2
  CZ Subsystem/1(CZ) -> Mux/3
  Mux/1 -> Cxyz/1
  Mx Subsystem/1(Mx) -> Mux1/1
  My Subsystem/1(My) -> Mux1/2
  Mux1/1 -> Mxyz/1
  Selector/1 -> Mz Subsystem/2(alpha), My Subsystem/5(alpha), Mx Subsystem/3(alpha), CZ Subsystem/2(alpha), CL Subsystem/1(alpha), CD/1  "alpha"
  Selector1/1 -> My Subsystem/1(Beta), Mx Subsystem/1(Beta), CZ Subsystem/1(beta)  "beta"

== system ASEToolBox2023a/Aerocraft Model/ACE Equation of 6DOF's Motion ==
  clock : Inport
  DeltXYZ : Inport  Port=2
  ACE Centroid Motion : Subsystem  mask(ACE Centroid Motion){}
      mask help: There is ACE Centroid Motion Model.
  ACE Mass Properties : Subsystem  mask(ACE Mass Properties){}
      mask help: There is ACE Mass Properties Model.
      mask Display:
      | %image(imread('aeromassprop.bmp','bmp'),'center');
      | port_label('input',1,'Time(s)','texmode','on');
      | port_label('output',1,'Mass(kg)','texmode','on');
  ACE Propulsion : Subsystem  mask(ACE Propulsion){}
      mask help: There is ACE Propulsion Model.
      mask Display:
      | %image(imread('aeropropulsion.bmp','bmp'),'center')
      | port_label('input',1,'Time(s)','texmode','on');
      | port_label('output',1,'P(N)','texmode','on');
  ACE Rotation Motion : Subsystem  mask(ACE Attitude Motion){}
      mask help: There is ACE Attitude Motion Model.
  Aero Force & Moment : Subsystem  InitFcn=|
      | if ~exist('dmassX','var')
      | dmassX = 0;              
      | end                      
      | if ~exist('dmassY','var')
      | dmassY = 0;              
      | end                      
      | if ~exist('dmassZ','var')
      | dmassZ = 0;              
      | end                      
      |                          
      | if ~exist('dCx','var')   
      | dCx = 0;                 
      | end                      
      | if ~exist('dCy','var')   
      | dCy = 0;                 
      | end                      
      | if ~exist('dCz','var')   
      | dCz = 0;                 
      | end                      
      |                          
      | if ~exist('dMx','var')   
      | dMx = 0;                 
      | end                      
      | if ~exist('dMy','var')   
      | dMy = 0;                 
      | end                      
      | if ~exist('dMz','var')   
      | dMz = 0;                 
      | end                      
      |                          
      | if ~exist('dp','var')    
      | dp = 0;                  
      | end
  Calculate H&S : Subsystem
  Constraint Equation2 : Subsystem  mask(Constraint Equation2){}
      mask help: There is Constraint Equation2 Model, which is used to calculate alpha beta and nu based on constraint equation.
  Ixyz : Constant  Value=[1.6 59.7 60.3]
  H : Outport
  theta : Outport  Port=2
  sigma : Outport  Port=3
  Vxyz : Outport  Port=4
  xyz : Outport  Port=5
  V : Outport  Port=6
  S : Outport  Port=7
  Eular : Outport  Port=8
  Wxyz1 : Outport  Port=9
  abv : Outport  Port=10
  static pressure : Outport  Port=11
  dynamic pressure : Outport  Port=12
  wires:
  Aero Force & Moment/4(dynamic pressure) -> dynamic pressure/1
  Aero Force & Moment/3(static pressure) -> static pressure/1
  ACE Centroid Motion/3(sigma) -> Constraint Equation2/2(sigma), sigma/1
  ACE Centroid Motion/5(V) -> V/1, Aero Force & Moment/4(V)
  ACE Centroid Motion/2(theta) -> Constraint Equation2/1(theta), theta/1
  DeltXYZ/1 -> Aero Force & Moment/2(DeltXYZ)
  Calculate H&S/1(H.) -> Aero Force & Moment/1(H), H/1
  Calculate H&S/2(S) -> S/1
  ACE Centroid Motion/1(xyz) -> xyz/1, Calculate H&S/1(xyz)
  Constraint Equation2/1(abv) -> abv/1, Aero Force & Moment/3(abv), ACE Centroid Motion/3(abv)
  Aero Force & Moment/2(Mxyz) -> ACE Rotation Motion/1(Mxyz)
  ACE Rotation Motion/1(Eular(deg)) -> Constraint Equation2/3(Eular), Eular/1
  ACE Rotation Motion/2(Wxyz1(deg/s)) -> Wxyz1/1, Aero Force & Moment/5(Wxyz)
  ACE Propulsion/1(P) -> ACE Centroid Motion/1(P)
  ACE Mass Properties/1(m) -> ACE Centroid Motion/2(m)
  Aero Force & Moment/1(F_aero) -> ACE Centroid Motion/4(F_aero)
  clock/1 -> ACE Mass Properties/1(Time), ACE Propulsion/1(Time)
  Ixyz/1 -> ACE Rotation Motion/2(Ixyz)
  ACE Centroid Motion/4(Vxyz) -> Vxyz/1
